simulink subsystem "CtrlEnv_Basic_refsub"  (R2025a)
settings: Solver=VariableStepAuto  StartTime=0.0  StopTime=10.0  RelTol=1e-3
settings Model: Creator=isaacito  LastModifiedBy=isaacito
settings SolverCC: AlgebraicLoopSolver=TrustRegion
settings OptimizationCC: ReuseModelBlockBuffer=off
settings DebuggingCC: UnconnectedInputMsg=warning  UnconnectedOutputMsg=warning  UnconnectedLineMsg=warning
settings ModelReferenceCC: EnableRefExpFcnMdlSchedulingChecks=on
settings RTWCC: GPUComputeCapability=3.5  DLArmComputeVersion=19.05

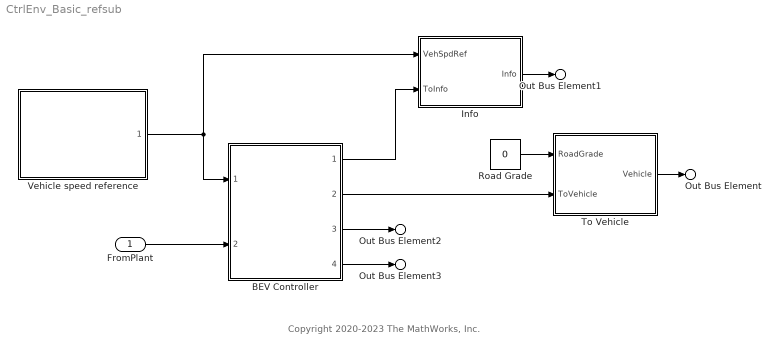
== system CtrlEnv_Basic_refsub ==
  note: Copyright 2020-2023 The MathWorks, Inc.
  FromPlant : Inport
  BEV Controller : Subsystem  ReferencedSubsystem=BEVController_Basic_refsub
      settings: OpenFcn=|
      | % Look under mask:
      | open_system(gcb, "force")
  Info : Subsystem
  Road Grade : Constant  Value=0
  To Vehicle : Subsystem
  Vehicle speed reference : Subsystem  ReferencedSubsystem=VehSpdRef_Basic_refsub
      settings: OpenFcn=|
      | % Look under mask:
      | open_system(gcb, "force")
  Out Bus Element : Outport  PortName=Inputs  Element=Vehicle
  Out Bus Element1 : Outport  PortName=Inputs  Element=Info
  Out Bus Element2 : Outport  PortName=Inputs  Element=MotorDrive
  Out Bus Element3 : Outport  PortName=Inputs  Element=BatteryHV
  wires:
  FromPlant/1 -> BEV Controller/2
  Road Grade/1 -> To Vehicle/1(RoadGrade)
  BEV Controller/2 -> To Vehicle/2(ToVehicle)
  To Vehicle/1(Vehicle) -> Out Bus Element/1
  BEV Controller/3 -> Out Bus Element2/1
  BEV Controller/4 -> Out Bus Element3/1
  BEV Controller/1 -> Info/2(ToInfo)
  Info/1(Info) -> Out Bus Element1/1
  Vehicle speed reference/1 -> BEV Controller/1, Info/1(VehSpdRef)

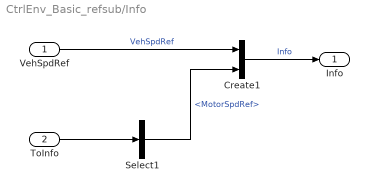
== system CtrlEnv_Basic_refsub/Info ==
  VehSpdRef : Inport
  ToInfo : Inport  Port=2
  Create1 : BusCreator  Inputs=2
  Select1 : BusSelector  OutputSignals=MotorSpdRef
  Info : Outport
  wires:
  ToInfo/1 -> Select1/1
  Create1/1 -> Info/1  "Info"
  Select1/1 -> Create1/2  "<MotorSpdRef>"
  VehSpdRef/1 -> Create1/1  "VehSpdRef"

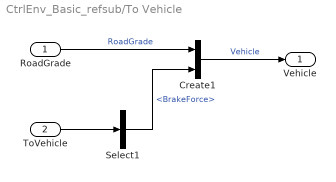
== system CtrlEnv_Basic_refsub/To Vehicle ==
  RoadGrade : Inport
  ToVehicle : Inport  Port=2
  Create1 : BusCreator  Inputs=2
  Select1 : BusSelector  OutputSignals=BrakeForce
  Vehicle : Outport
  wires:
  Create1/1 -> Vehicle/1  "Vehicle"
  ToVehicle/1 -> Select1/1
  RoadGrade/1 -> Create1/1  "RoadGrade"
  Select1/1 -> Create1/2  "<BrakeForce>"
